simulink model "all_sc_0001_0193"  (R2026a)
settings: Solver=VariableStepAuto  StopTime=40  FixedStep=0.1  MaxStep=.1
model workspace (MAT data in the model file):
  T = [0 0.05 0.1 0.15 0.2 0.25 0.3 0.35 0.4 0.45 0.5 0.55 ... (701 elements, 701x1)]
  U = [3.99594136536 3.99594136536 3.99594136536 3.99594136536 3.99594136536 3.99594136536 3.99594136536 3.99594136536 3.99594136536 3.99594136536 3.99594136536 3.99594136536 ... (701 elements, 701x1)]
undefined symbols (not defined in the file): A, B, C, Dd
(part 1 of 3)
settings Model: Creator=syaghoub  LastModifiedBy=harry_31916
settings DataIOCC: ExternalInput=simin

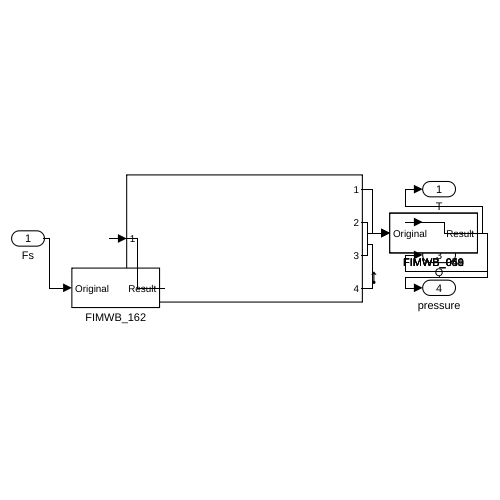
[thumbnail: Simulink's stored preview of the top-level diagram]
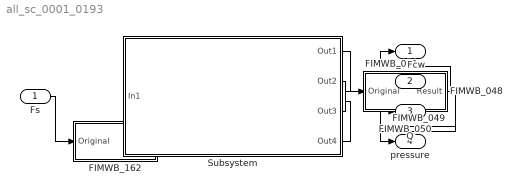
== system all_sc_0001_0193 ==
  Fs : Inport
  FIMWB_048 : Subsystem  Tag=fimwb.fault.48
  FIMWB_049 : Subsystem  Tag=fimwb.fault.49
  FIMWB_050 : Subsystem  Tag=fimwb.fault.50
  FIMWB_051 : Subsystem  Tag=fimwb.fault.51
  FIMWB_162 : Subsystem  Tag=fimwb.fault.162
  Subsystem : Subsystem
  T : Outport  VectorParamsAs1DForOutWhenUnconnected=off
  Fcw : Outport  Port=2  VectorParamsAs1DForOutWhenUnconnected=off
  Q : Outport  Port=3  VectorParamsAs1DForOutWhenUnconnected=off
  pressure : Outport  Port=4  VectorParamsAs1DForOutWhenUnconnected=off
  wires:
  Subsystem/1(Out1) -> FIMWB_048/1(Original)
  FIMWB_048/1(Result) -> T/1
  Subsystem/2(Out2) -> FIMWB_049/1(Original)
  FIMWB_049/1(Result) -> Fcw/1
  Subsystem/3(Out3) -> FIMWB_050/1(Original)
  FIMWB_050/1(Result) -> Q/1
  Subsystem/4(Out4) -> FIMWB_051/1(Original)
  FIMWB_051/1(Result) -> pressure/1
  Fs/1 -> FIMWB_162/1(Original)
  FIMWB_162/1(Result) -> Subsystem/1(In1)

== system all_sc_0001_0193/FIMWB_048 ==
  Original : Inport
  Result : Outport
  wires:
  Original/1 -> Result/1

== system all_sc_0001_0193/FIMWB_049 ==
  Original : Inport
  Result : Outport
  wires:
  Original/1 -> Result/1

== system all_sc_0001_0193/FIMWB_050 ==
  Original : Inport
  Result : Outport
  wires:
  Original/1 -> Result/1

== system all_sc_0001_0193/FIMWB_051 ==
  Original : Inport
  Result : Outport
  wires:
  Original/1 -> Result/1

== system all_sc_0001_0193/FIMWB_162 ==
  Original : Inport
  Result : Outport
  wires:
  Original/1 -> Result/1

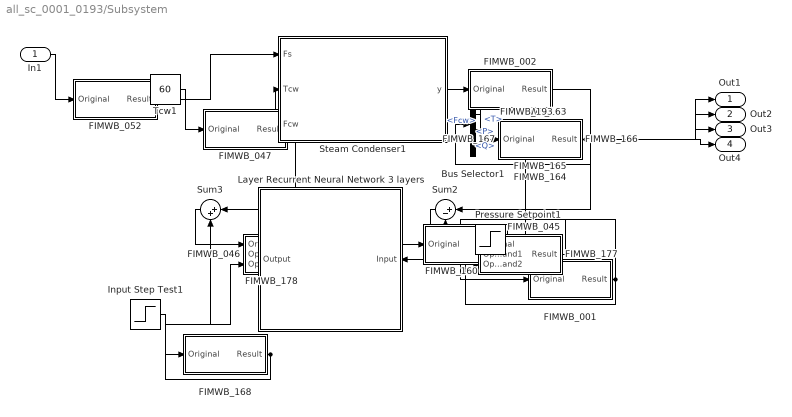
== system all_sc_0001_0193/Subsystem ==
  In1 : Inport
  Bus Selector1 : BusSelector  OutputSignals=T,Fcw,Q,P
  FIMWB_001 : Subsystem  Tag=fimwb.fault.1
  FIMWB_002 : Subsystem  Tag=fimwb.fault.2
  FIMWB_045 : Subsystem  Tag=fimwb.fault.45
  FIMWB_046 : Subsystem  Tag=fimwb.fault.46
  FIMWB_047 : Subsystem  Tag=fimwb.fault.47
  FIMWB_052 : Subsystem  Tag=fimwb.fault.52
  FIMWB_160 : Subsystem  Tag=fimwb.fault.160
  FIMWB_163 : Subsystem  Tag=fimwb.fault.163
  FIMWB_164 : Subsystem  Tag=fimwb.fault.164
  FIMWB_165 : Subsystem  Tag=fimwb.fault.165
  FIMWB_166 : Subsystem  Tag=fimwb.fault.166
  FIMWB_167 : Subsystem  Tag=fimwb.fault.167
  FIMWB_168 : Subsystem  Tag=fimwb.fault.168
  FIMWB_177 : Subsystem  Tag=fimwb.fault.177
  FIMWB_178 : Subsystem  Tag=fimwb.fault.178
  FIMWB_193 : Subsystem  Tag=fimwb.fault.193
  Input Step Test1 : Step  Time=10  FinalValue=0  SampleTime=0
  "Layer Recurrent Neural Network 3 layers " : Subsystem  mask{ai_layer_1_delayed_1=[0;0;0], ai_layer_1_delayed_2=[0;0;0], Parameter3=[]}
      mask prompts: ai_layer_1_delayed_1 "Initial layer 1 state at timestep 0."; ai_layer_1_delayed_2 "Initial layer 1 state at timestep -1."
      mask help: Layer Recurrent Neural Network
      mask Display: e = 0.06;c1 = [120 150 230]/255;c2 = ([120 150 230]+0)/383;c3 = ([120 150 230]+128)/383;patch([0 1 1 0],[0 0 1 1],c1);patch([0 1 1 1-e 1-e 0+e],[0 0 1 1-e 0+e 0+e],c2);patch([0 0 1 1-e 0+e 0+e],[0 1 1 1-e 1-e 0+e],c3);plot([0 1 1 0 0],[0 0 1 1 0]);fprintf('NNET');port_label('input',1,' Input');port_label('output',1,'Output ');
  Pressure Setpoint1 : Step  Time=2  InitialValue=90  FinalValue=87  SampleTime=0
  Steam Condenser1 : Subsystem  mask{V=3, Mcw=500, UA=356.972413581334, tau=1, Fcw=107.8880952381, P=90, T=80}
      mask prompts: V "Volume [m3]"; Mcw "CW Holdup [kg]"; UA "UA [kW/K]"; tau "Actuator time constant [s]"; Fcw "Fcw [kg/s]"; P "P [kPa]"; T "T [degC]"
      mask init:
      | y1=[.3 .3 .7 .7 .3 NaN .4 .4 NaN .5 .5 NaN .6 .6 NaN 0.2 0.3 NaN 0.7 0.8 NaN 0.7 0.8 NaN 0.82 NaN 0.18];
      | x1=[.8 .2 .2 .8 .8 NaN .8 .2 NaN .8 .2 NaN .8 .2 NaN 0.5 0.5 NaN 0.3 0.3 NaN 0.7 0.7 NaN -0.05 NaN 1.05];
      | y2=0.3:0.05:0.7;
      | x2=sqrt(0.0625-(y2-0.5).^2);
      | y3=[.5 .5 .8 NaN 0.2 0.4 0.4];
      | x3=[x2(5)+0.65 0.95 0.95 NaN .1 .1 0.35-x2(3)];
      mask Display:
      | plot([x1 NaN 0.65+x2 NaN 0.35-x2 NaN x3],[y1 NaN y2 NaN y2 NaN y3])
      | port_label('input',1,'Fs')
      | port_label('input',2,'Tcw')
      | port_label('input',3,'Fcw')
      | port_label('output',1,'y')
  Sum2 : Sum  Inputs=|+-  InputSameDT=on  OutDataTypeStr=Inherit: Same as first input
  Sum3 : Sum  Inputs=|++  InputSameDT=on  OutDataTypeStr=Inherit: Same as first input
  Tcw1 : Constant  Value=60  VectorParams1D=off
  Out1 : Outport  VectorParamsAs1DForOutWhenUnconnected=off
  Out2 : Outport  Port=2  VectorParamsAs1DForOutWhenUnconnected=off
  Out3 : Outport  Port=3  VectorParamsAs1DForOutWhenUnconnected=off
  Out4 : Outport  Port=4  VectorParamsAs1DForOutWhenUnconnected=off
  wires:
  Sum2/1 -> FIMWB_177/1(Original)
  Sum3/1 -> FIMWB_178/1(Original)
  Bus Selector1/4 -> FIMWB_193/1(Original)  "<P>"
  FIMWB_193/1(Result) -> FIMWB_166/1(Original), FIMWB_167/1(Original)
  Pressure Setpoint1/1 -> FIMWB_001/1(Original)
  FIMWB_001/1(Result) -> Sum2/2, FIMWB_177/3(Operand2)
  Steam Condenser1/1(y) -> FIMWB_002/1(Original)
  FIMWB_002/1(Result) -> Bus Selector1/1
  FIMWB_177/1(Result) -> FIMWB_045/1(Original)
  FIMWB_045/1(Result) -> "Layer Recurrent Neural Network 3 layers "/1(Input)
  FIMWB_178/1(Result) -> FIMWB_046/1(Original)
  FIMWB_046/1(Result) -> Steam Condenser1/3(Fcw)
  Tcw1/1 -> FIMWB_047/1(Original)
  FIMWB_047/1(Result) -> Steam Condenser1/2(Tcw)
  In1/1 -> FIMWB_052/1(Original)
  FIMWB_052/1(Result) -> Steam Condenser1/1(Fs)
  "Layer Recurrent Neural Network 3 layers "/1(Output) -> FIMWB_160/1(Original)
  FIMWB_160/1(Result) -> Sum3/1, FIMWB_178/2(Operand1)
  Bus Selector1/1 -> FIMWB_163/1(Original)  "<T>"
  FIMWB_163/1(Result) -> Out1/1
  Bus Selector1/2 -> FIMWB_164/1(Original)  "<Fcw>"
  FIMWB_164/1(Result) -> Out2/1
  Bus Selector1/3 -> FIMWB_165/1(Original)  "<Q>"
  FIMWB_165/1(Result) -> Out3/1
  FIMWB_166/1(Result) -> Sum2/1, FIMWB_177/2(Operand1)
  FIMWB_167/1(Result) -> Out4/1
  Input Step Test1/1 -> FIMWB_168/1(Original)
  FIMWB_168/1(Result) -> Sum3/2, FIMWB_178/3(Operand2)

== system all_sc_0001_0193/Subsystem/FIMWB_001 ==
  Original : Inport
  Result : Outport
  wires:
  Original/1 -> Result/1

== system all_sc_0001_0193/Subsystem/FIMWB_002 ==
  Original : Inport
  Result : Outport
  wires:
  Original/1 -> Result/1

== system all_sc_0001_0193/Subsystem/FIMWB_045 ==
  Original : Inport
  Result : Outport
  wires:
  Original/1 -> Result/1

== system all_sc_0001_0193/Subsystem/FIMWB_046 ==
  Original : Inport
  Result : Outport
  wires:
  Original/1 -> Result/1

== system all_sc_0001_0193/Subsystem/FIMWB_047 ==
  Original : Inport
  Result : Outport
  wires:
  Original/1 -> Result/1

== system all_sc_0001_0193/Subsystem/FIMWB_052 ==
  Original : Inport
  Result : Outport
  wires:
  Original/1 -> Result/1

== system all_sc_0001_0193/Subsystem/FIMWB_160 ==
  Original : Inport
  Result : Outport
  wires:
  Original/1 -> Result/1

== system all_sc_0001_0193/Subsystem/FIMWB_163 ==
  Original : Inport
  Result : Outport
  wires:
  Original/1 -> Result/1

== system all_sc_0001_0193/Subsystem/FIMWB_164 ==
  Original : Inport
  Result : Outport
  wires:
  Original/1 -> Result/1

== system all_sc_0001_0193/Subsystem/FIMWB_165 ==
  Original : Inport
  Result : Outport
  wires:
  Original/1 -> Result/1

== system all_sc_0001_0193/Subsystem/FIMWB_166 ==
  Original : Inport
  Result : Outport
  wires:
  Original/1 -> Result/1

== system all_sc_0001_0193/Subsystem/FIMWB_167 ==
  Original : Inport
  Result : Outport
  wires:
  Original/1 -> Result/1

== system all_sc_0001_0193/Subsystem/FIMWB_168 ==
  Original : Inport
  Result : Outport
  wires:
  Original/1 -> Result/1

== system all_sc_0001_0193/Subsystem/FIMWB_177 ==
  Original : Inport
  Operand1 : Inport  Port=2
  Operand2 : Inport  Port=3
  Unused2 : Terminator
  Unused3 : Terminator
  Result : Outport
  wires:
  Original/1 -> Result/1
  Operand1/1 -> Unused2/1
  Operand2/1 -> Unused3/1

== system all_sc_0001_0193/Subsystem/FIMWB_178 ==
  Original : Inport
  Operand1 : Inport  Port=2
  Operand2 : Inport  Port=3
  Unused2 : Terminator
  Unused3 : Terminator
  Result : Outport
  wires:
  Original/1 -> Result/1
  Operand1/1 -> Unused2/1
  Operand2/1 -> Unused3/1

== system all_sc_0001_0193/Subsystem/FIMWB_193 ==
  Original : Inport
  Result : Outport
  wires:
  Original/1 -> Result/1

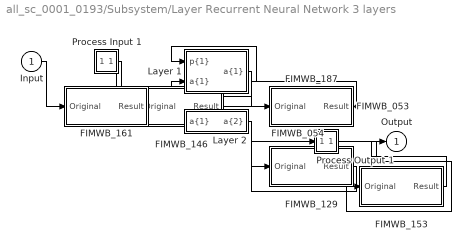
== system all_sc_0001_0193/Subsystem/Layer Recurrent Neural Network 3 layers  ==
  Input : Inport  PortDimensions=1
      mask Display: e = 0.06;c1 = [120 230 180]/255;c2 = ([120 230 180]+0)/(256+128);c3 = ([120 230 180]+128)/(256+128);patch([0 1 1 0],[0 0 1 1],c1);patch([0 1 1 1-e 1-e 0+e],[0 0 1 1-e 0+e 0+e],c2);patch([0 0 1 1-e 0+e 0+e],[0 1 1 1-e 1-e 0+e],c3);plot([0 1 1 0 0],[0 0 1 1 0]);
  FIMWB_053 : Subsystem  Tag=fimwb.fault.53
  FIMWB_054 : Subsystem  Tag=fimwb.fault.54
  FIMWB_129 : Subsystem  Tag=fimwb.fault.129
  FIMWB_146 : Subsystem  Tag=fimwb.fault.146
  FIMWB_153 : Subsystem  Tag=fimwb.fault.153
  FIMWB_161 : Subsystem  Tag=fimwb.fault.161
  FIMWB_187 : Subsystem  Tag=fimwb.fault.187
  Layer 1 : Subsystem
      mask Display: e = 0.06;c1 = [120 150 230]/255;c2 = ([120 150 230]+0)/383;c3 = ([120 150 230]+128)/383;patch([0 1 1 0],[0 0 1 1],c1);patch([0 1 1 1-e 1-e 0+e],[0 0 1 1-e 0+e 0+e],c2);patch([0 0 1 1-e 0+e 0+e],[0 1 1 1-e 1-e 0+e],c3);plot([0 1 1 0 0],[0 0 1 1 0]);
  Layer 2 : Subsystem
      mask Display: e = 0.06;c1 = [120 150 230]/255;c2 = ([120 150 230]+0)/383;c3 = ([120 150 230]+128)/383;patch([0 1 1 0],[0 0 1 1],c1);patch([0 1 1 1-e 1-e 0+e],[0 0 1 1-e 0+e 0+e],c2);patch([0 0 1 1-e 0+e 0+e],[0 1 1 1-e 1-e 0+e],c3);plot([0 1 1 0 0],[0 0 1 1 0]);
  Process Input 1 : Subsystem
      mask Display: e = 0.06;c1 = [120 150 230]/255;c2 = ([120 150 230]+0)/383;c3 = ([120 150 230]+128)/383;patch([0 1 1 0],[0 0 1 1],c1);patch([0 1 1 1-e 1-e 0+e],[0 0 1 1-e 0+e 0+e],c2);patch([0 0 1 1-e 0+e 0+e],[0 1 1 1-e 1-e 0+e],c3);plot([0 1 1 0 0],[0 0 1 1 0]);
  Process Output 1 : Subsystem
      mask Display: e = 0.06;c1 = [120 150 230]/255;c2 = ([120 150 230]+0)/383;c3 = ([120 150 230]+128)/383;patch([0 1 1 0],[0 0 1 1],c1);patch([0 1 1 1-e 1-e 0+e],[0 0 1 1-e 0+e 0+e],c2);patch([0 0 1 1-e 0+e 0+e],[0 1 1 1-e 1-e 0+e],c3);plot([0 1 1 0 0],[0 0 1 1 0]);
  Output : Outport  InitialOutput=0  VectorParamsAs1DForOutWhenUnconnected=off
      mask Display: e = 0.06;c1 = [120 230 180]/255;c2 = ([120 230 180]+0)/(256+128);c3 = ([120 230 180]+128)/(256+128);patch([0 1 1 0],[0 0 1 1],c1);patch([0 1 1 1-e 1-e 0+e],[0 0 1 1-e 0+e 0+e],c2);patch([0 0 1 1-e 0+e 0+e],[0 1 1 1-e 1-e 0+e],c3);plot([0 1 1 0 0],[0 0 1 1 0]);
  wires:
  Layer 1/1("a{1}") -> FIMWB_187/1(Original)
  FIMWB_187/1(Result) -> FIMWB_053/1(Original), FIMWB_054/1(Original)
  FIMWB_053/1(Result) -> Layer 1/2("a{1} ")
  FIMWB_054/1(Result) -> Layer 2/1("a{1} ")
  Layer 2/1("a{2}") -> FIMWB_129/1(Original)
  FIMWB_129/1(Result) -> Process Output 1/1(a)
  Process Input 1/1(p) -> FIMWB_146/1(Original)
  FIMWB_146/1(Result) -> Layer 1/1("p{1}")
  Process Output 1/1(y) -> FIMWB_153/1(Original)
  FIMWB_153/1(Result) -> Output/1
  Input/1 -> FIMWB_161/1(Original)
  FIMWB_161/1(Result) -> Process Input 1/1(x)

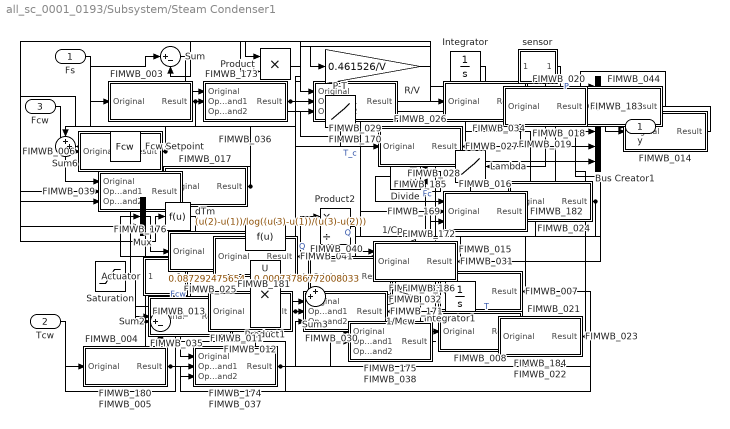
== system all_sc_0001_0193/Subsystem/Steam Condenser1 ==
  Fs : Inport
  Tcw : Inport  Port=2
  Fcw : Inport  Port=3
  1/Cp : Gain  Gain=1/4.2  OutDataTypeStr=Inherit: Same as input  ParamDataTypeStr=Inherit: Same as input
  1/Mcw : Gain  Gain=1/Mcw  OutDataTypeStr=Inherit: Same as input  ParamDataTypeStr=Inherit: Same as input
  Actuator : Subsystem  mask(Transfer Function with Initial Outputs){N=[1], D=[tau 1], Y0=Fcw, U0=Fcw}
      mask prompts: N "SimulinkBlocks:simulink_extras:Numerator_MP"; D "SimulinkBlocks:simulink_extras:Denominator_MP"; Y0 "SimulinkBlocks:simulink_extras:InitialOutput_MP"; U0 "SimulinkBlocks:simulink_extras:InitialInput_MP"
      mask help: SimulinkBlocks:simulink_extras:TransferFunctionWithInitialOutputs_MD
      mask init:
      | [A,B,C,Dd]=tf2ss(N,D);
      | if (isempty(Y0));
      |     [m,n]=size(C);
      |     Y0=zeros(1,m); 
      | end; 
      | if (isempty(U0));
      |     [m,p]=size(B);
      |     U0=zeros(1,p);
      | end;
      | X0=getxo(A,B,C,Dd,U0,Y0,0);
      mask Help: Specify the initial output for the transfer function.  An optimization routine attempts to determine the appropriate initial states so that the specified initial output is achieved.  For more details, see the m-file getxo.m
      mask Display:
      | if(isempty(N) || isempty(D))
      | disp('H(s)')
      | else
      | dpoly(N,D,'s')
      | end
  Bus Creator1 : BusCreator  Inputs=6
  Divide : Product  Inputs=/*  InputSameDT=on  RndMeth=Zero  OutDataTypeStr=Inherit: Same as first input
  FIMWB_003 : Subsystem  Tag=fimwb.fault.3
  FIMWB_004 : Subsystem  Tag=fimwb.fault.4
  FIMWB_005 : Subsystem  Tag=fimwb.fault.5
  FIMWB_006 : Subsystem  Tag=fimwb.fault.6
  FIMWB_007 : Subsystem  Tag=fimwb.fault.7
  FIMWB_008 : Subsystem  Tag=fimwb.fault.8
  FIMWB_011 : Subsystem  Tag=fimwb.fault.11
  FIMWB_012 : Subsystem  Tag=fimwb.fault.12
  FIMWB_013 : Subsystem  Tag=fimwb.fault.13
  FIMWB_014 : Subsystem  Tag=fimwb.fault.14
  FIMWB_015 : Subsystem  Tag=fimwb.fault.15
  FIMWB_016 : Subsystem  Tag=fimwb.fault.16
  FIMWB_017 : Subsystem  Tag=fimwb.fault.17
  FIMWB_018 : Subsystem  Tag=fimwb.fault.18
  FIMWB_019 : Subsystem  Tag=fimwb.fault.19
  FIMWB_020 : Subsystem  Tag=fimwb.fault.20
  FIMWB_021 : Subsystem  Tag=fimwb.fault.21
  FIMWB_022 : Subsystem  Tag=fimwb.fault.22
  FIMWB_023 : Subsystem  Tag=fimwb.fault.23
  FIMWB_024 : Subsystem  Tag=fimwb.fault.24
  FIMWB_025 : Subsystem  Tag=fimwb.fault.25
  FIMWB_026 : Subsystem  Tag=fimwb.fault.26
  FIMWB_027 : Subsystem  Tag=fimwb.fault.27
  FIMWB_028 : Subsystem  Tag=fimwb.fault.28
  FIMWB_029 : Subsystem  Tag=fimwb.fault.29
  FIMWB_030 : Subsystem  Tag=fimwb.fault.30
  FIMWB_031 : Subsystem  Tag=fimwb.fault.31
  FIMWB_032 : Subsystem  Tag=fimwb.fault.32
  FIMWB_033 : Subsystem  Tag=fimwb.fault.33
  FIMWB_034 : Subsystem  Tag=fimwb.fault.34
  FIMWB_035 : Subsystem  Tag=fimwb.fault.35
  FIMWB_036 : Subsystem  Tag=fimwb.fault.36
  FIMWB_037 : Subsystem  Tag=fimwb.fault.37
  FIMWB_038 : Subsystem  Tag=fimwb.fault.38
  FIMWB_039 : Subsystem  Tag=fimwb.fault.39
  FIMWB_040 : Subsystem  Tag=fimwb.fault.40
  FIMWB_041 : Subsystem  Tag=fimwb.fault.41
  FIMWB_044 : Subsystem  Tag=fimwb.fault.44
  FIMWB_169 : Subsystem  Tag=fimwb.fault.169
  FIMWB_170 : Subsystem  Tag=fimwb.fault.170
  FIMWB_171 : Subsystem  Tag=fimwb.fault.171
  FIMWB_172 : Subsystem  Tag=fimwb.fault.172
  FIMWB_173 : Subsystem  Tag=fimwb.fault.173
  FIMWB_174 : Subsystem  Tag=fimwb.fault.174
  FIMWB_175 : Subsystem  Tag=fimwb.fault.175
  FIMWB_176 : Subsystem  Tag=fimwb.fault.176
  FIMWB_180 : Subsystem  Tag=fimwb.fault.180
  FIMWB_181 : Subsystem  Tag=fimwb.fault.181
  FIMWB_182 : Subsystem  Tag=fimwb.fault.182
  FIMWB_183 : Subsystem  Tag=fimwb.fault.183
  FIMWB_184 : Subsystem  Tag=fimwb.fault.184
  FIMWB_185 : Subsystem  Tag=fimwb.fault.185
  FIMWB_186 : Subsystem  Tag=fimwb.fault.186
  Fcw Setpoint : Constant  Value=Fcw
  Integrator : Integrator  InitialCondition=P
  Integrator1 : Integrator  InitialCondition=T
  Lambda : Lookup  InputValues=[50 60 70 80 90 100 110]  Table=[2305.42 2293.64 2283.30 2274.05 2265.65 2257.92 2250.76]
  Mux : Mux  Inputs=3
  P-T : Lookup  InputValues=[50 60 70 80 90 100 110]  Table=[81.3167 85.9258 89.9315 93.4854 96.6870 99.6059 102.2923]
  Product : Product  InputSameDT=on  RndMeth=Zero  OutDataTypeStr=Inherit: Same as first input
  Product1 : Product  InputSameDT=on  RndMeth=Zero  OutDataTypeStr=Inherit: Same as first input
  Product2 : Product  Inputs=*/  InputSameDT=on  RndMeth=Zero  OutDataTypeStr=Inherit: Same as first input
  R/V : Gain  Gain=0.461526/V  OutDataTypeStr=Inherit: Same as input  ParamDataTypeStr=Inherit: Same as input
  Saturation : Saturate  UpperLimit=200  LowerLimit=0
  Sum : Sum  Inputs=|+-  InputSameDT=on  OutDataTypeStr=Inherit: Same as first input
  Sum2 : Sum  Inputs=|+-  InputSameDT=on  OutDataTypeStr=Inherit: Same as first input
  Sum3 : Sum  Inputs=++|  InputSameDT=on  OutDataTypeStr=Inherit: Same as first input
  Sum6 : Sum  Inputs=|++  InputSameDT=on  OutDataTypeStr=Inherit: Same as first input
  U : Fcn  Expr=0.0872924756541668/u^0.8+0.00073786772008033
  dTm : Fcn  Expr=(u(2)-u(1))/log((u(3)-u(1))/(u(3)-u(2)))
  sensor : Subsystem  mask(Transfer Function with Initial Outputs){N=[1], D=[tau/2 1], Y0=P, U0=P}
      mask prompts: N "SimulinkBlocks:simulink_extras:Numerator_MP"; D "SimulinkBlocks:simulink_extras:Denominator_MP"; Y0 "SimulinkBlocks:simulink_extras:InitialOutput_MP"; U0 "SimulinkBlocks:simulink_extras:InitialInput_MP"
      mask help: SimulinkBlocks:simulink_extras:TransferFunctionWithInitialOutputs_MD
      mask init:
      | [A,B,C,Dd]=tf2ss(N,D);
      | if (isempty(Y0));
      |     [m,n]=size(C);
      |     Y0=zeros(1,m); 
      | end; 
      | if (isempty(U0));
      |     [m,p]=size(B);
      |     U0=zeros(1,p);
      | end;
      | X0=getxo(A,B,C,Dd,U0,Y0,0);
      mask Help: Specify the initial output for the transfer function.  An optimization routine attempts to determine the appropriate initial states so that the specified initial output is achieved.  For more details, see the m-file getxo.m
      mask Display:
      | if(isempty(N) || isempty(D))
      | disp('H(s)')
      | else
      | dpoly(N,D,'s')
      | end
  y : Outport  VectorParamsAs1DForOutWhenUnconnected=off
  wires:
  Divide/1 -> FIMWB_169/1(Original)  "Fc"
  Product/1 -> FIMWB_170/1(Original)
  Product1/1 -> FIMWB_171/1(Original)
  Product2/1 -> FIMWB_172/1(Original)  "Q"
  Sum/1 -> FIMWB_173/1(Original)
  Sum2/1 -> FIMWB_174/1(Original)
  Sum3/1 -> FIMWB_175/1(Original)
  Sum6/1 -> FIMWB_176/1(Original)
  Tcw/1 -> FIMWB_180/1(Original)
  FIMWB_180/1(Result) -> FIMWB_004/1(Original), FIMWB_005/1(Original)
  Actuator/1(Out1) -> FIMWB_181/1(Original)  "Fcw"
  FIMWB_181/1(Result) -> FIMWB_011/1(Original), FIMWB_012/1(Original), FIMWB_013/1(Original)
  FIMWB_169/1(Result) -> FIMWB_182/1(Original)
  FIMWB_182/1(Result) -> FIMWB_015/1(Original), FIMWB_016/1(Original)
  Integrator/1 -> FIMWB_183/1(Original)
  FIMWB_183/1(Result) -> FIMWB_018/1(Original), FIMWB_019/1(Original), FIMWB_020/1(Original)
  Integrator1/1 -> FIMWB_184/1(Original)  "T"
  FIMWB_184/1(Result) -> FIMWB_021/1(Original), FIMWB_022/1(Original), FIMWB_023/1(Original)
  P-T/1 -> FIMWB_185/1(Original)  "T_c"
  FIMWB_185/1(Result) -> FIMWB_026/1(Original), FIMWB_027/1(Original), FIMWB_028/1(Original)
  FIMWB_172/1(Result) -> FIMWB_186/1(Original)
  FIMWB_186/1(Result) -> FIMWB_031/1(Original), FIMWB_032/1(Original), FIMWB_033/1(Original)
  Fs/1 -> FIMWB_003/1(Original)
  FIMWB_003/1(Result) -> Sum/1, FIMWB_173/2(Operand1)
  FIMWB_004/1(Result) -> Mux/1
  FIMWB_005/1(Result) -> Sum2/1, FIMWB_174/2(Operand1)
  Fcw/1 -> FIMWB_006/1(Original)
  FIMWB_006/1(Result) -> Sum6/1, FIMWB_176/2(Operand1)
  1/Cp/1 -> FIMWB_007/1(Original)
  FIMWB_007/1(Result) -> Sum3/1, FIMWB_175/2(Operand1)
  1/Mcw/1 -> FIMWB_008/1(Original)
  FIMWB_008/1(Result) -> Integrator1/1
  FIMWB_011/1(Result) -> Bus Creator1/6
  FIMWB_012/1(Result) -> Product1/1, FIMWB_171/2(Operand1)
  FIMWB_013/1(Result) -> U/1
  Bus Creator1/1 -> FIMWB_014/1(Original)
  FIMWB_014/1(Result) -> y/1
  FIMWB_015/1(Result) -> Bus Creator1/3
  FIMWB_016/1(Result) -> Sum/2, FIMWB_173/3(Operand2)
  Fcw Setpoint/1 -> FIMWB_017/1(Original)
  FIMWB_017/1(Result) -> Sum6/2, FIMWB_176/3(Operand2)
  FIMWB_018/1(Result) -> Lambda/1
  FIMWB_019/1(Result) -> P-T/1
  FIMWB_020/1(Result) -> sensor/1(In1)
  FIMWB_021/1(Result) -> Bus Creator1/5
  FIMWB_022/1(Result) -> Mux/2
  FIMWB_023/1(Result) -> Sum2/2, FIMWB_174/3(Operand2)
  Lambda/1 -> FIMWB_024/1(Original)
  FIMWB_024/1(Result) -> Divide/1, FIMWB_169/2(Operand1)
  Mux/1 -> FIMWB_025/1(Original)
  FIMWB_025/1(Result) -> dTm/1
  FIMWB_026/1(Result) -> Bus Creator1/2
  FIMWB_027/1(Result) -> Mux/3
  FIMWB_028/1(Result) -> Product/2, FIMWB_170/3(Operand2)
  FIMWB_170/1(Result) -> FIMWB_029/1(Original)
  FIMWB_029/1(Result) -> R/V/1
  FIMWB_171/1(Result) -> FIMWB_030/1(Original)
  FIMWB_030/1(Result) -> Sum3/2, FIMWB_175/3(Operand2)
  FIMWB_031/1(Result) -> 1/Cp/1
  FIMWB_032/1(Result) -> Bus Creator1/4
  FIMWB_033/1(Result) -> Divide/2, FIMWB_169/3(Operand2)
  R/V/1 -> FIMWB_034/1(Original)
  FIMWB_034/1(Result) -> Integrator/1
  Saturation/1 -> FIMWB_035/1(Original)
  FIMWB_035/1(Result) -> Actuator/1(In1)
  FIMWB_173/1(Result) -> FIMWB_036/1(Original)
  FIMWB_036/1(Result) -> Product/1, FIMWB_170/2(Operand1)
  FIMWB_174/1(Result) -> FIMWB_037/1(Original)
  FIMWB_037/1(Result) -> Product1/2, FIMWB_171/3(Operand2)
  FIMWB_175/1(Result) -> FIMWB_038/1(Original)
  FIMWB_038/1(Result) -> 1/Mcw/1
  FIMWB_176/1(Result) -> FIMWB_039/1(Original)
  FIMWB_039/1(Result) -> Saturation/1
  U/1 -> FIMWB_040/1(Original)  "Q"
  FIMWB_040/1(Result) -> Product2/2, FIMWB_172/3(Operand2)
  dTm/1 -> FIMWB_041/1(Original)
  FIMWB_041/1(Result) -> Product2/1, FIMWB_172/2(Operand1)
  sensor/1(Out1) -> FIMWB_044/1(Original)  "P"
  FIMWB_044/1(Result) -> Bus Creator1/1

== system all_sc_0001_0193/Subsystem/Layer Recurrent Neural Network 3 layers /FIMWB_053 ==
  Original : Inport
  Result : Outport
  wires:
  Original/1 -> Result/1

== system all_sc_0001_0193/Subsystem/Layer Recurrent Neural Network 3 layers /FIMWB_054 ==
  Original : Inport
  Result : Outport
  wires:
  Original/1 -> Result/1

== system all_sc_0001_0193/Subsystem/Layer Recurrent Neural Network 3 layers /FIMWB_129 ==
  Original : Inport
  Result : Outport
  wires:
  Original/1 -> Result/1

== system all_sc_0001_0193/Subsystem/Layer Recurrent Neural Network 3 layers /FIMWB_146 ==
  Original : Inport
  Result : Outport
  wires:
  Original/1 -> Result/1

== system all_sc_0001_0193/Subsystem/Layer Recurrent Neural Network 3 layers /FIMWB_153 ==
  Original : Inport
  Result : Outport
  wires:
  Original/1 -> Result/1

== system all_sc_0001_0193/Subsystem/Layer Recurrent Neural Network 3 layers /FIMWB_161 ==
  Original : Inport
  Result : Outport
  wires:
  Original/1 -> Result/1

== system all_sc_0001_0193/Subsystem/Layer Recurrent Neural Network 3 layers /FIMWB_187 ==
  Original : Inport
  Result : Outport
  wires:
  Original/1 -> Result/1

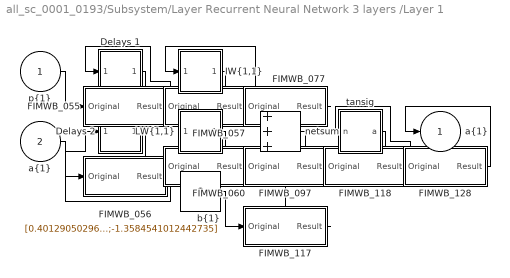
== system all_sc_0001_0193/Subsystem/Layer Recurrent Neural Network 3 layers /Layer 1 ==
  "p{1}" : Inport  PortDimensions=1
      mask Display: e = 0.06;c1 = [120 230 180]/255;c2 = ([120 230 180]+0)/(256+128);c3 = ([120 230 180]+128)/(256+128);patch([0 1 1 0],[0 0 1 1],c1);patch([0 1 1 1-e 1-e 0+e],[0 0 1 1-e 0+e 0+e],c2);patch([0 0 1 1-e 0+e 0+e],[0 1 1 1-e 1-e 0+e],c3);plot([0 1 1 0 0],[0 0 1 1 0]);
  "a{1} " : Inport  Port=2  PortDimensions=3
      mask Display: e = 0.06;c1 = [120 230 180]/255;c2 = ([120 230 180]+0)/(256+128);c3 = ([120 230 180]+128)/(256+128);patch([0 1 1 0],[0 0 1 1],c1);patch([0 1 1 1-e 1-e 0+e],[0 0 1 1-e 0+e 0+e],c2);patch([0 0 1 1-e 0+e 0+e],[0 1 1 1-e 1-e 0+e],c3);plot([0 1 1 0 0],[0 0 1 1 0]);
  Delays 1 : Subsystem
      mask Display: e = 0.06;c1 = [120 150 230]/255;c2 = ([120 150 230]+0)/383;c3 = ([120 150 230]+128)/383;patch([0 1 1 0],[0 0 1 1],c1);patch([0 1 1 1-e 1-e 0+e],[0 0 1 1-e 0+e 0+e],c2);patch([0 0 1 1-e 0+e 0+e],[0 1 1 1-e 1-e 0+e],c3);plot([0 1 1 0 0],[0 0 1 1 0]);disp('0');
  Delays 2 : Subsystem
      mask Display: e = 0.06;c1 = [120 150 230]/255;c2 = ([120 150 230]+0)/383;c3 = ([120 150 230]+128)/383;patch([0 1 1 0],[0 0 1 1],c1);patch([0 1 1 1-e 1-e 0+e],[0 0 1 1-e 0+e 0+e],c2);patch([0 0 1 1-e 0+e 0+e],[0 1 1 1-e 1-e 0+e],c3);plot([0 1 1 0 0],[0 0 1 1 0]);disp('1-2');
  FIMWB_055 : Subsystem  Tag=fimwb.fault.55
  FIMWB_056 : Subsystem  Tag=fimwb.fault.56
  FIMWB_057 : Subsystem  Tag=fimwb.fault.57
  FIMWB_060 : Subsystem  Tag=fimwb.fault.60
  FIMWB_077 : Subsystem  Tag=fimwb.fault.77
  FIMWB_097 : Subsystem  Tag=fimwb.fault.97
  FIMWB_117 : Subsystem  Tag=fimwb.fault.117
  FIMWB_118 : Subsystem  Tag=fimwb.fault.118
  FIMWB_128 : Subsystem  Tag=fimwb.fault.128
  "IW{1,1}" : Subsystem
      mask Display: e = 0.06;c1 = [120 150 230]/255;c2 = ([120 150 230]+0)/383;c3 = ([120 150 230]+128)/383;patch([0 1 1 0],[0 0 1 1],c1);patch([0 1 1 1-e 1-e 0+e],[0 0 1 1-e 0+e 0+e],c2);patch([0 0 1 1-e 0+e 0+e],[0 1 1 1-e 1-e 0+e],c3);plot([0 1 1 0 0],[0 0 1 1 0]);disp('W');
  "LW{1,1}" : Subsystem
      mask Display: e = 0.06;c1 = [120 150 230]/255;c2 = ([120 150 230]+0)/383;c3 = ([120 150 230]+128)/383;patch([0 1 1 0],[0 0 1 1],c1);patch([0 1 1 1-e 1-e 0+e],[0 0 1 1-e 0+e 0+e],c2);patch([0 0 1 1-e 0+e 0+e],[0 1 1 1-e 1-e 0+e],c3);plot([0 1 1 0 0],[0 0 1 1 0]);disp('W');
  "b{1}" : Constant  Value=[0.40129050296348601;-0.12475735064274925;-1.3584541012442735]
      mask Display: e = 0.06;c1 = [120 150 230]/255;c2 = ([120 150 230]+0)/383;c3 = ([120 150 230]+128)/383;patch([0 1 1 0],[0 0 1 1],c1);patch([0 1 1 1-e 1-e 0+e],[0 0 1 1-e 0+e 0+e],c2);patch([0 0 1 1-e 0+e 0+e],[0 1 1 1-e 1-e 0+e],c3);plot([0 1 1 0 0],[0 0 1 1 0]);disp('b');
  netsum : Sum  Inputs=3  InputSameDT=on  SaturateOnIntegerOverflow=on  OutDataTypeStr=Inherit: Same as first input
      mask Display: e = 0.06;c1 = [120 150 230]/255;c2 = ([120 150 230]+0)/383;c3 = ([120 150 230]+128)/383;patch([0 1 1 0],[0 0 1 1],c1);patch([0 1 1 1-e 1-e 0+e],[0 0 1 1-e 0+e 0+e],c2);patch([0 0 1 1-e 0+e 0+e],[0 1 1 1-e 1-e 0+e],c3);plot([0 1 1 0 0],[0 0 1 1 0]);disp('+');
  tansig : Subsystem  mask(TANSIG){}
      mask help: nnet:Simulink:TansigBlockDesc
      mask init:
      | network;
      mask Help: helpview([docroot '/deeplearning/ref/tansig.html']);
      mask Display:
      | e = 0.06;
      | c1 = [120 150 230]/255;
      | c2 = ([120 150 230]+0)/383;
      | c3 = ([120 150 230]+128)/383;
      | patch([0 1 1 0],[0 0 1 1],c1);
      | patch([0 1 1 1-e 1-e 0+e],[0 0 1 1-e 0+e 0+e],c2);
      | patch([0 0 1 1-e 0+e 0+e],[0 1 1 1-e 1-e 0+e],c3);
      | color('white')
      | plot([-1 1]*0.35+0.5,[0 0]+0.5)
      | plot([0 0]+0.5,[-1 1]*0.35+0.5)
      | color('black')
      | xx = -1:0.01:1;
      | plot(xx*0.35+0.5,1./(1+exp(-5*xx))*0.7+0.15)
      | plot([0 1 1 0 0],[0 0 1 1 0])
  "a{1}" : Outport  InitialOutput=[0;0;0]  VectorParamsAs1DForOutWhenUnconnected=off
      mask Display: e = 0.06;c1 = [120 230 180]/255;c2 = ([120 230 180]+0)/(256+128);c3 = ([120 230 180]+128)/(256+128);patch([0 1 1 0],[0 0 1 1],c1);patch([0 1 1 1-e 1-e 0+e],[0 0 1 1-e 0+e 0+e],c2);patch([0 0 1 1-e 0+e 0+e],[0 1 1 1-e 1-e 0+e],c3);plot([0 1 1 0 0],[0 0 1 1 0]);
  wires:
  "p{1}"/1 -> FIMWB_055/1(Original)
  FIMWB_055/1(Result) -> Delays 1/1("p{1}")
  "a{1} "/1 -> FIMWB_056/1(Original)
  FIMWB_056/1(Result) -> Delays 2/1("p{1}")
  Delays 1/1("pd{1,1}") -> FIMWB_057/1(Original)
  FIMWB_057/1(Result) -> "IW{1,1}"/1("pd{1,1}")
  Delays 2/1("pd{1,1}") -> FIMWB_060/1(Original)
  FIMWB_060/1(Result) -> "LW{1,1}"/1("ad{1,1}")
  "IW{1,1}"/1("iz{1,1}") -> FIMWB_077/1(Original)
  FIMWB_077/1(Result) -> netsum/1
  "LW{1,1}"/1("lz{1,1}") -> FIMWB_097/1(Original)
  FIMWB_097/1(Result) -> netsum/2
  "b{1}"/1 -> FIMWB_117/1(Original)
  FIMWB_117/1(Result) -> netsum/3
  netsum/1 -> FIMWB_118/1(Original)
  FIMWB_118/1(Result) -> tansig/1(n)
  tansig/1(a) -> FIMWB_128/1(Original)
  FIMWB_128/1(Result) -> "a{1}"/1

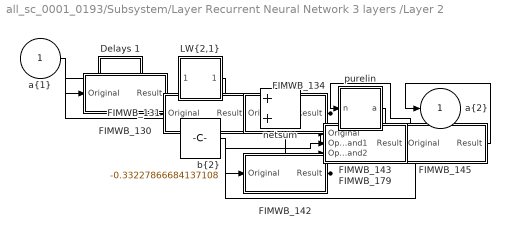
== system all_sc_0001_0193/Subsystem/Layer Recurrent Neural Network 3 layers /Layer 2 ==
  "a{1} " : Inport  PortDimensions=3
      mask Display: e = 0.06;c1 = [120 230 180]/255;c2 = ([120 230 180]+0)/(256+128);c3 = ([120 230 180]+128)/(256+128);patch([0 1 1 0],[0 0 1 1],c1);patch([0 1 1 1-e 1-e 0+e],[0 0 1 1-e 0+e 0+e],c2);patch([0 0 1 1-e 0+e 0+e],[0 1 1 1-e 1-e 0+e],c3);plot([0 1 1 0 0],[0 0 1 1 0]);
  Delays 1 : Subsystem
      mask Display: e = 0.06;c1 = [120 150 230]/255;c2 = ([120 150 230]+0)/383;c3 = ([120 150 230]+128)/383;patch([0 1 1 0],[0 0 1 1],c1);patch([0 1 1 1-e 1-e 0+e],[0 0 1 1-e 0+e 0+e],c2);patch([0 0 1 1-e 0+e 0+e],[0 1 1 1-e 1-e 0+e],c3);plot([0 1 1 0 0],[0 0 1 1 0]);disp('0');
  FIMWB_130 : Subsystem  Tag=fimwb.fault.130
  FIMWB_131 : Subsystem  Tag=fimwb.fault.131
  FIMWB_134 : Subsystem  Tag=fimwb.fault.134
  FIMWB_142 : Subsystem  Tag=fimwb.fault.142
  FIMWB_143 : Subsystem  Tag=fimwb.fault.143
  FIMWB_145 : Subsystem  Tag=fimwb.fault.145
  FIMWB_179 : Subsystem  Tag=fimwb.fault.179
  "LW{2,1}" : Subsystem
      mask Display: e = 0.06;c1 = [120 150 230]/255;c2 = ([120 150 230]+0)/383;c3 = ([120 150 230]+128)/383;patch([0 1 1 0],[0 0 1 1],c1);patch([0 1 1 1-e 1-e 0+e],[0 0 1 1-e 0+e 0+e],c2);patch([0 0 1 1-e 0+e 0+e],[0 1 1 1-e 1-e 0+e],c3);plot([0 1 1 0 0],[0 0 1 1 0]);disp('W');
  "b{2}" : Constant  Value=-0.33227866684137108
      mask Display: e = 0.06;c1 = [120 150 230]/255;c2 = ([120 150 230]+0)/383;c3 = ([120 150 230]+128)/383;patch([0 1 1 0],[0 0 1 1],c1);patch([0 1 1 1-e 1-e 0+e],[0 0 1 1-e 0+e 0+e],c2);patch([0 0 1 1-e 0+e 0+e],[0 1 1 1-e 1-e 0+e],c3);plot([0 1 1 0 0],[0 0 1 1 0]);disp('b');
  netsum : Sum  Inputs=2  InputSameDT=on  SaturateOnIntegerOverflow=on  OutDataTypeStr=Inherit: Same as first input
      mask Display: e = 0.06;c1 = [120 150 230]/255;c2 = ([120 150 230]+0)/383;c3 = ([120 150 230]+128)/383;patch([0 1 1 0],[0 0 1 1],c1);patch([0 1 1 1-e 1-e 0+e],[0 0 1 1-e 0+e 0+e],c2);patch([0 0 1 1-e 0+e 0+e],[0 1 1 1-e 1-e 0+e],c3);plot([0 1 1 0 0],[0 0 1 1 0]);disp('+');
  purelin : Subsystem  mask(PURELIN){}
      mask help: nnet:Simulink:PurelinBlockDesc
      mask init:
      | network;
      mask Help: helpview([docroot '/deeplearning/ref/purelin.html']);
      mask Display:
      | e = 0.06;
      | c1 = [120 150 230]/255;
      | c2 = ([120 150 230]+0)/383;
      | c3 = ([120 150 230]+128)/383;
      | patch([0 1 1 0],[0 0 1 1],c1);
      | patch([0 1 1 1-e 1-e 0+e],[0 0 1 1-e 0+e 0+e],c2);
      | patch([0 0 1 1-e 0+e 0+e],[0 1 1 1-e 1-e 0+e],c3);
      | color('white')
      | plot([-1 1]*0.35+0.5,[0 0]+0.5)
      | plot([0 0]+0.5,[-1 1]*0.35+0.5)
      | color('black')
      | plot([-1 1]*0.35+0.5,[-1 1]*0.35+0.5)
      | plot([0 1 1 0 0],[0 0 1 1 0])
  "a{2}" : Outport  InitialOutput=0  VectorParamsAs1DForOutWhenUnconnected=off
      mask Display: e = 0.06;c1 = [120 230 180]/255;c2 = ([120 230 180]+0)/(256+128);c3 = ([120 230 180]+128)/(256+128);patch([0 1 1 0],[0 0 1 1],c1);patch([0 1 1 1-e 1-e 0+e],[0 0 1 1-e 0+e 0+e],c2);patch([0 0 1 1-e 0+e 0+e],[0 1 1 1-e 1-e 0+e],c3);plot([0 1 1 0 0],[0 0 1 1 0]);
  wires:
  netsum/1 -> FIMWB_179/1(Original)
  "a{1} "/1 -> FIMWB_130/1(Original)
  FIMWB_130/1(Result) -> Delays 1/1("p{2}")
  Delays 1/1("pd{2,1}") -> FIMWB_131/1(Original)
  FIMWB_131/1(Result) -> "LW{2,1}"/1("ad{2,1}")
  "LW{2,1}"/1("lz{2,1}") -> FIMWB_134/1(Original)
  FIMWB_134/1(Result) -> netsum/1, FIMWB_179/2(Operand1)
  "b{2}"/1 -> FIMWB_142/1(Original)
  FIMWB_142/1(Result) -> netsum/2, FIMWB_179/3(Operand2)
  FIMWB_179/1(Result) -> FIMWB_143/1(Original)
  FIMWB_143/1(Result) -> purelin/1(n)
  purelin/1(a) -> FIMWB_145/1(Original)
  FIMWB_145/1(Result) -> "a{2}"/1

== system all_sc_0001_0193/Subsystem/Layer Recurrent Neural Network 3 layers /Process Input 1 ==
  x : Inport  PortDimensions=1
      mask Display: e = 0.06;c1 = [120 230 180]/255;c2 = ([120 230 180]+0)/(256+128);c3 = ([120 230 180]+128)/(256+128);patch([0 1 1 0],[0 0 1 1],c1);patch([0 1 1 1-e 1-e 0+e],[0 0 1 1-e 0+e 0+e],c2);patch([0 0 1 1-e 0+e 0+e],[0 1 1 1-e 1-e 0+e],c3);plot([0 1 1 0 0],[0 0 1 1 0]);
  FIMWB_147 : Subsystem  Tag=fimwb.fault.147
  FIMWB_152 : Subsystem  Tag=fimwb.fault.152
  mapminmax : Subsystem  mask(MAPMINMAX Preprocess){xmin=-3.7742393716738434, xmax=5.7997431225043385, ymin=-1, ymax=1}
      mask prompts: xmin "nnet:Simulink:MinX"; xmax "nnet:Simulink:MaxX"; ymin "nnet:Simulink:MinY"; ymax "nnet:Simulink:MaxY"
      mask help: nnet:Simulink:MapminmaxBlockDesc
      mask init:
      | network;
      mask Help: helpview([docroot '/deeplearning/ref/mapminmax.html']);
      mask DialogControl xmin Prompt: Minimum X (Nx1 column)
      mask DialogControl xmax Prompt: Maximum X (Nx1 column)
      mask DialogControl ymin Prompt: Minimum Y
      mask DialogControl ymax Prompt: Maximum Y
      mask Display:
      | e = 0.06;
      | c1 = [120 150 230]/255;
      | c2 = ([120 150 230]+0)/383;
      | c3 = ([120 150 230]+128)/383;
      | patch([0 1 1 0],[0 0 1 1],c1);
      | patch([0 1 1 1-e 1-e 0+e],[0 0 1 1-e 0+e 0+e],c2);
      | patch([0 0 1 1-e 0+e 0+e],[0 1 1 1-e 1-e 0+e],c3);
      | plot([0 1 1 0 0],[0 0 1 1 0])
      | port_label('input',1,'x')
      | port_label('output',1,'y')
  p : Outport  PortDimensions=1  VectorParamsAs1DForOutWhenUnconnected=off
      mask Display: e = 0.06;c1 = [120 230 180]/255;c2 = ([120 230 180]+0)/(256+128);c3 = ([120 230 180]+128)/(256+128);patch([0 1 1 0],[0 0 1 1],c1);patch([0 1 1 1-e 1-e 0+e],[0 0 1 1-e 0+e 0+e],c2);patch([0 0 1 1-e 0+e 0+e],[0 1 1 1-e 1-e 0+e],c3);plot([0 1 1 0 0],[0 0 1 1 0]);
  wires:
  x/1 -> FIMWB_147/1(Original)
  FIMWB_147/1(Result) -> mapminmax/1(x)
  mapminmax/1(y) -> FIMWB_152/1(Original)
  FIMWB_152/1(Result) -> p/1

== system all_sc_0001_0193/Subsystem/Layer Recurrent Neural Network 3 layers /Process Output 1 ==
  a : Inport  PortDimensions=1
      mask Display: e = 0.06;c1 = [120 230 180]/255;c2 = ([120 230 180]+0)/(256+128);c3 = ([120 230 180]+128)/(256+128);patch([0 1 1 0],[0 0 1 1],c1);patch([0 1 1 1-e 1-e 0+e],[0 0 1 1-e 0+e 0+e],c2);patch([0 0 1 1-e 0+e 0+e],[0 1 1 1-e 1-e 0+e],c3);plot([0 1 1 0 0],[0 0 1 1 0]);
  FIMWB_154 : Subsystem  Tag=fimwb.fault.154
  FIMWB_159 : Subsystem  Tag=fimwb.fault.159
  mapminmax_reverse : Subsystem  mask(MAPMINMAX Reverse Process){xmin=-30.855068745036114, xmax=66.879264965962932, ymin=-1, ymax=1}
      mask prompts: xmin "nnet:Simulink:MinX"; xmax "nnet:Simulink:MaxX"; ymin "nnet:Simulink:MinY"; ymax "nnet:Simulink:MaxY"
      mask help: nnet:Simulink:MapminmaxreverseBlockDesc
      mask init:
      | network;
      mask Help: helpview([docroot '/deeplearning/ref/mapminmax.html']);
      mask DialogControl xmin Prompt: Minimum X (Nx1 column)
      mask DialogControl xmax Prompt: Maximum X (Nx1 column)
      mask DialogControl ymin Prompt: Minimum Y
      mask DialogControl ymax Prompt: Maximum Y
      mask Display:
      | e = 0.06;
      | c1 = [120 150 230]/255;
      | c2 = ([120 150 230]+0)/383;
      | c3 = ([120 150 230]+128)/383;
      | patch([0 1 1 0],[0 0 1 1],c1);
      | patch([0 1 1 1-e 1-e 0+e],[0 0 1 1-e 0+e 0+e],c2);
      | patch([0 0 1 1-e 0+e 0+e],[0 1 1 1-e 1-e 0+e],c3);
      | plot([0 1 1 0 0],[0 0 1 1 0])
      | port_label('input',1,'y')
      | port_label('output',1,'x')
  y : Outport  PortDimensions=1  VectorParamsAs1DForOutWhenUnconnected=off
      mask Display: e = 0.06;c1 = [120 230 180]/255;c2 = ([120 230 180]+0)/(256+128);c3 = ([120 230 180]+128)/(256+128);patch([0 1 1 0],[0 0 1 1],c1);patch([0 1 1 1-e 1-e 0+e],[0 0 1 1-e 0+e 0+e],c2);patch([0 0 1 1-e 0+e 0+e],[0 1 1 1-e 1-e 0+e],c3);plot([0 1 1 0 0],[0 0 1 1 0]);
  wires:
  a/1 -> FIMWB_154/1(Original)
  FIMWB_154/1(Result) -> mapminmax_reverse/1(y)
  mapminmax_reverse/1(x) -> FIMWB_159/1(Original)
  FIMWB_159/1(Result) -> y/1

== system all_sc_0001_0193/Subsystem/Steam Condenser1/Actuator ==
  In1 : Inport
  FIMWB_009 : Subsystem  Tag=fimwb.fault.9
  FIMWB_010 : Subsystem  Tag=fimwb.fault.10
  State Space : StateSpace  A=A  B=B  C=C  D=Dd  InitialCondition=X0
  Out1 : Outport  InitialOutput=0  VectorParamsAs1DForOutWhenUnconnected=off
  wires:
  In1/1 -> FIMWB_009/1(Original)
  FIMWB_009/1(Result) -> State Space/1
  State Space/1 -> FIMWB_010/1(Original)
  FIMWB_010/1(Result) -> Out1/1

== system all_sc_0001_0193/Subsystem/Steam Condenser1/FIMWB_003 ==
  Original : Inport
  Result : Outport
  wires:
  Original/1 -> Result/1

== system all_sc_0001_0193/Subsystem/Steam Condenser1/FIMWB_004 ==
  Original : Inport
  Result : Outport
  wires:
  Original/1 -> Result/1

== system all_sc_0001_0193/Subsystem/Steam Condenser1/FIMWB_005 ==
  Original : Inport
  Result : Outport
  wires:
  Original/1 -> Result/1

== system all_sc_0001_0193/Subsystem/Steam Condenser1/FIMWB_006 ==
  Original : Inport
  Result : Outport
  wires:
  Original/1 -> Result/1

== system all_sc_0001_0193/Subsystem/Steam Condenser1/FIMWB_007 ==
  Original : Inport
  Result : Outport
  wires:
  Original/1 -> Result/1

== system all_sc_0001_0193/Subsystem/Steam Condenser1/FIMWB_008 ==
  Original : Inport
  Result : Outport
  wires:
  Original/1 -> Result/1
